simulink model "hrg_wa_v10_2_port_bench"  (R2025a)
settings: Solver=FixedStepDiscrete  StartTime=0.0  StopTime=p.duration  FixedStep=p.Ts  RelTol=1e-3
model workspace (MAT data in the model file):
  Ad = [0.987688405123 5.68131323296e-08 -982.899001209 0.00680633562581 0 0 943869.866875 -6.2854468604 113668107.931 -505.246320907 62170953.3395 -882829.706009 ... (144 elements, 12x12)]
  Bd = [1.07541978092e-16 2.15044631223e-18 1.17750014529e-11 2.35440509738e-13 0.71349520314 0 -1.10105605369e-08 -2.20157780066e-10 -9.65252715165e-07 -1.93016562843e-08 -4.58609339763e-07 -2.49830556256e-09 ... (24 elements, 12x2)]
  bench_input = [0 2.5e-05 5e-05 7.5e-05 0.0001 0.000125 0.00015 0.000175 0.0002 0.000225 0.00025 0.000275 ... (3603 elements, 1201x3)]
  c : object (value not decoded)
  p : object (value not decoded)
  x0 = [2.76318298201e-12; 1.16825502693e-12; 0; 0; 0; 0; 0; 0; 0; 0; 0; 0]
symbols that are objects in the model workspace (value not decoded): p
libraries: hrg_wa_v10_2_modules x5
(part 2 of 2)

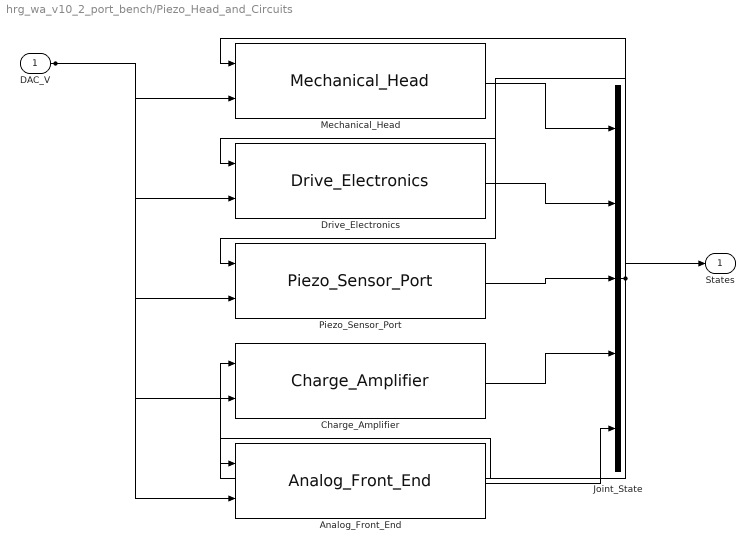
== system hrg_wa_v10_2_port_bench/Piezo_Head_and_Circuits ==
  DAC_V : Inport
  Analog_Front_End : hrg_wa_v10_2_modules/Analog_Front_End  SystemSampleTime=-1  VariantActivationTime=update diagram  EmptyChoice=off  PassThrough=off  PassThroughVariantControl=(default)  EmptyChoiceVariantControl=(default)  AllowFlexibleInterface=on  Latency=0  AutoFrameSizeCalculation=off
  Charge_Amplifier : hrg_wa_v10_2_modules/Charge_Amplifier  SystemSampleTime=-1  VariantActivationTime=update diagram  EmptyChoice=off  PassThrough=off  PassThroughVariantControl=(default)  EmptyChoiceVariantControl=(default)  AllowFlexibleInterface=on  Latency=0  AutoFrameSizeCalculation=off
  Drive_Electronics : hrg_wa_v10_2_modules/Drive_Electronics  SystemSampleTime=-1  VariantActivationTime=update diagram  EmptyChoice=off  PassThrough=off  PassThroughVariantControl=(default)  EmptyChoiceVariantControl=(default)  AllowFlexibleInterface=on  Latency=0  AutoFrameSizeCalculation=off
  Joint_State : Mux  Inputs=5
  Mechanical_Head : hrg_wa_v10_2_modules/Mechanical_Head  SystemSampleTime=-1  VariantActivationTime=update diagram  EmptyChoice=off  PassThrough=off  PassThroughVariantControl=(default)  EmptyChoiceVariantControl=(default)  AllowFlexibleInterface=on  Latency=0  AutoFrameSizeCalculation=off
  Piezo_Sensor_Port : hrg_wa_v10_2_modules/Piezo_Sensor_Port  SystemSampleTime=-1  VariantActivationTime=update diagram  EmptyChoice=off  PassThrough=off  PassThroughVariantControl=(default)  EmptyChoiceVariantControl=(default)  AllowFlexibleInterface=on  Latency=0  AutoFrameSizeCalculation=off
  States : Outport
  wires:
  Joint_State/1 -> Mechanical_Head/1, Drive_Electronics/1, Piezo_Sensor_Port/1, Charge_Amplifier/1, Analog_Front_End/1, States/1
  DAC_V/1 -> Mechanical_Head/2, Drive_Electronics/2, Piezo_Sensor_Port/2, Charge_Amplifier/2, Analog_Front_End/2
  Mechanical_Head/1 -> Joint_State/1
  Drive_Electronics/1 -> Joint_State/2
  Piezo_Sensor_Port/1 -> Joint_State/3
  Charge_Amplifier/1 -> Joint_State/4
  Analog_Front_End/1 -> Joint_State/5
